simulink model "ADCS_Simulink_FSW"  (R2025b)
settings: Solver=VariableStepAuto  StartTime=8000  StopTime=8700  FixedStep=0.001  RelTol=1e-3
PreLoadFcn:
  | addpath(genpath('../'))
  | adcsModelSetup();
values from neighbouring files (symbols this model uses):
  dT_Control = 1/10    (= 0.1)    [adcsModelSetup.m]
  fNoiseOn = 0    [adcsModelSetup.m]
undefined symbols (not defined in the file or in its folder): DiscIntNeverNeededParam, IAU, juliandate
libraries: vrlib x16, simulink_extras x7, sharedtransform x5, sharedutil x4, aerolibutil x4, sFunctionLibrary x4, simulink x3, matrix_library x2, aerolibtransform2 x2
(part 2 of 2)

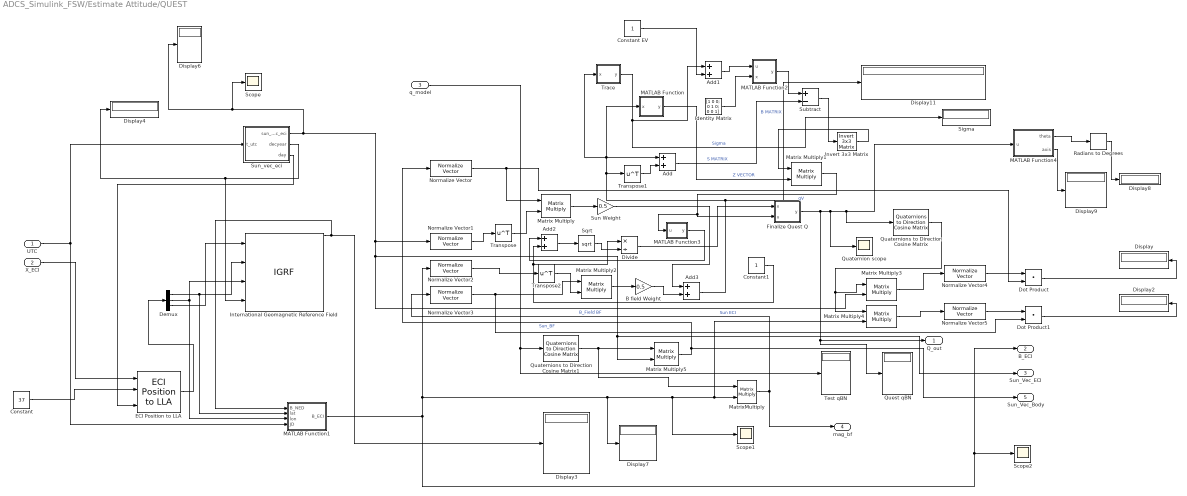
== system ADCS_Simulink_FSW/Estimate Attitude/QUEST ==
  UTC : Inport
  X_ECI : Inport  Port=2
  q_model : Inport  Port=3
  Add{,1..3} (4 alike) : Sum
  B field Weight : Gain  Gain=0.5
  Constant : Constant  Value=37
  Constant EV : Constant
  Constant1 : Constant
  Demux : Demux  Outputs=3
  Display{,2..4,6..9,11} (9 alike) : Display
  Divide : Product  Inputs=*/
  Dot Product : DotProduct  OutDataTypeStr=Inherit: Inherit via internal rule
  Dot Product1 : DotProduct  OutDataTypeStr=Inherit: Inherit via internal rule
  ECI Position to LLA : aerolibtransform2/ECI Position to LLA  red=IAU-2000/2006  year=2013  month=January  day=1  hour=0  min=0  sec=0  deltaT=Day  errorflag=Error  extraparamflag=on  eunits=Metric (MKS)  earthmodel=WGS84  flat=1/298.257223563  eqradius=6378137
      settings: AttributesFormatString=%<red>
  Finalize Quest Q : MATLAB Function  TreatAsAtomicUnit=on
  Identity Matrix : Constant  Value=[1 0 0; 0 1 0; 0 0 1]
  International Geomagnetic Reference Field : IGRF  month=January  day=1  year=2020
      settings: AttributesFormatString=%<generation>
  Invert 3x3 Matrix : aerolibutil/Invert  3x3 Matrix
  MATLAB Function : MATLAB Function  TreatAsAtomicUnit=on
  MATLAB Function1 : MATLAB Function  TreatAsAtomicUnit=on
  MATLAB Function2 : MATLAB Function  TreatAsAtomicUnit=on
  MATLAB Function3 : MATLAB Function  TreatAsAtomicUnit=on
  MATLAB Function4 : MATLAB Function  TreatAsAtomicUnit=on
  Matrix Multiply{,1..5} (6 alike) : Product  Multiplication=Matrix(*)
  MatrixMultiply : Product  Multiplication=Matrix(*)
  Normalize Vector{,1..5} (6 alike) : vrlib/Utilities/Normalize Vector  maxzero=0
  Quaternion scope : Scope
      settings: ActiveDisplayYMinimum=-1.3373181480846994  ActiveDisplayYMaximum=1.336803706475939
  Quaternions to Direction Cosine Matrix : sharedtransform/Quaternions to  Direction Cosine Matrix  aMode=aMode
  Quaternions to Direction Cosine Matrix1 : sharedtransform/Quaternions to  Direction Cosine Matrix  aMode=aMode
  Quest qBN : Display
  Radians to Degrees : simulink_extras/Transformations/Radians to Degrees
  Scope : Scope
      settings: ActiveDisplayYMinimum=-1.0754499109455182  ActiveDisplayYMaximum=0.0072133154143029787
  Scope1 : Scope
      settings: ActiveDisplayYMinimum=-1  ActiveDisplayYMaximum=1  DataLoggingVariableName=ScopeData2
  Scope2 : Scope
      settings: ActiveDisplayYMinimum=-2220.8584339639051  ActiveDisplayYMaximum=7667.7859361134633  DataLoggingVariableName=ScopeData26
  Sigma : Display
  Sqrt : Sqrt
  Subtract : Sum  Inputs=+-
  Sun Weight : Gain  Gain=0.5
  Sun_vec_eci : MATLAB Function  TreatAsAtomicUnit=on
  Test qBN : Display
  Trace : MATLAB Function  TreatAsAtomicUnit=on
  Transpose : Math  Operator=transpose
  Transpose1 : Math  Operator=transpose
  Transpose2 : Math  Operator=transpose
  Q_out : Outport
  B_ECI : Outport  Port=2
  Sun_Vec_ECI : Outport  Port=3
  mag_bf : Outport  Port=4
  Sun_Vec_Body : Outport  Port=5
  wires:
  Sun_vec_eci/3(day) -> ECI Position to LLA/6
  MATLAB Function4/1(theta) -> Radians to Degrees/1
  Finalize Quest Q/1(y) -> Quest qBN/1, Q_out/1, MATLAB Function4/1(u), Quaternions to Direction Cosine Matrix/1, Quaternion scope/1
  Normalize Vector4/1 -> Dot Product/1
  Normalize Vector3/1 -> Matrix Multiply2/1, Dot Product1/2
  Transpose2/1 -> Matrix Multiply2/2
  Normalize Vector1/1 -> Transpose/1
  Normalize Vector5/1 -> Dot Product1/1
  ECI Position to LLA/1 -> Demux/1
  Constant/1 -> ECI Position to LLA/3
  Constant1/1 -> Add2/2, Divide/1
  q_model/1 -> Quaternions to Direction Cosine Matrix1/1, Test qBN/1
  Dot Product/1 -> Display/1
  Sun_vec_eci/1(sun_vec_eci) -> Display6/1, Scope/1, Sun_Vec_ECI/1, Matrix Multiply5/2, Matrix Multiply3/2, Normalize Vector1/1  "Sun ECI"
  Matrix Multiply/1 -> Sun Weight/1
  Demux/1 -> International Geomagnetic Reference Field/2, MATLAB Function1/2(lat)
  Radians to Degrees/1 -> Display8/1
  MatrixMultiply/1 -> Normalize Vector3/1, mag_bf/1  "B_Field BF"
  Quaternions to Direction Cosine Matrix/1 -> Matrix Multiply4/1, Matrix Multiply3/1
  Matrix Multiply5/1 -> Sun_Vec_Body/1, Normalize Vector/1  "Sun_BF"
  Invert 3x3 Matrix/1 -> Matrix Multiply1/1
  Sqrt/1 -> Divide/2
  Demux/3 -> International Geomagnetic Reference Field/1
  Transpose/1 -> Matrix Multiply/2
  Transpose1/1 -> Add/2
  Identity Matrix/1 -> MATLAB Function2/2(x)
  Matrix Multiply3/1 -> Normalize Vector4/1
  Quaternions to Direction Cosine Matrix1/1 -> MatrixMultiply/1, Matrix Multiply5/1
  International Geomagnetic Reference Field/1 -> MATLAB Function1/1(B_NED), Display3/1
  Dot Product1/1 -> Display2/1
  Subtract/1 -> Invert 3x3 Matrix/1
  UTC/1 -> Sun_vec_eci/1(t_utc), MATLAB Function1/4(JD)
  Demux/2 -> MATLAB Function1/3(lon), International Geomagnetic Reference Field/3
  Matrix Multiply2/1 -> B field Weight/1
  Trace/1(y) -> Sigma/1, Add1/1  "Sigma"
  Add/1 -> Subtract/2  "S MATRIX"
  Add2/1 -> Sqrt/1
  MATLAB Function/1(y) -> Matrix Multiply1/2  "Z VECTOR"
  Divide/1 -> Finalize Quest Q/1(x)
  Sun_vec_eci/2(decyear) -> Display4/1, International Geomagnetic Reference Field/4
  Matrix Multiply1/1 -> MATLAB Function3/1(u), Finalize Quest Q/2(u)  "qV"
  X_ECI/1 -> ECI Position to LLA/1
  MATLAB Function2/1(y) -> Subtract/1
  Sun Weight/1 -> Add3/1
  MATLAB Function4/2(axis) -> Display9/1
  Matrix Multiply4/1 -> Normalize Vector5/1
  B field Weight/1 -> Add3/2
  Normalize Vector2/1 -> Transpose2/1
  Add3/1 -> Display11/1, Transpose1/1, MATLAB Function/1(x), Trace/1(x), Add/1  "B MATRIX"
  Add1/1 -> MATLAB Function2/1(u)
  MATLAB Function3/1(y) -> Add2/1
  Normalize Vector/1 -> Matrix Multiply/1, Dot Product/2
  Constant EV/1 -> Add1/2
  MATLAB Function1/1(B_ECI) -> Normalize Vector2/1, MatrixMultiply/2, Matrix Multiply4/2, Scope1/1, Display7/1, Scope2/1, B_ECI/1

== system ADCS_Simulink_FSW/Estimate Attitude/WhiteNoise ==
  Band-Limited White Noise : simulink/Sources/Band-Limited White Noise  Cov=NoisePower  Ts=dT  seed=randi([0 1000],size(NoisePower))
  Data Type Conversion6 : DataTypeConversion  OutDataTypeStr=single  SaturateOnIntegerOverflow=off  RndMeth=Floor
  Out1 : Outport
  wires:
  Band-Limited White Noise/1 -> Data Type Conversion6/1
  Data Type Conversion6/1 -> Out1/1

== system ADCS_Simulink_FSW/NoiseAndDiscretise/GaussianNoise ==
  Data Type Conversion6 : DataTypeConversion  OutDataTypeStr=single  SaturateOnIntegerOverflow=off  RndMeth=Floor
  Random Number : RandomNumber  Mean=Mean  Variance=Variance  Seed=randi([0 1000],size(Variance))  SampleTime=dT  VectorParams1D=off
  Out1 : Outport
  wires:
  Random Number/1 -> Data Type Conversion6/1
  Data Type Conversion6/1 -> Out1/1

== matlab function ADCS_Simulink_FSW/Angle Error ==
  data: u input; y output
function y = fcn(u)
    a = u(1);
    
    y = 2 * acos(a);
end

== matlab function ADCS_Simulink_FSW/Create Desired Quaternion/Calc Angle ==
  data: u input; angle output
function angle = fcn(u)

angle=acos((trace(u)-1)/2);

== matlab function ADCS_Simulink_FSW/Create Desired Quaternion/Calc Axis of rotation ==
  data: a input; y output; b input
function y = fcn(a,b)

y = 1/(2*sin(a))*[b(3,2)-b(2,3); b(1,3)-b(3,1); b(2,1)-b(1,2)];

== matlab function ADCS_Simulink_FSW/Estimate Attitude/QUEST/MATLAB Function ==
  data: x input; y output
function y = fcn(x)
y=ones(3,1);
y(1)=x(2,3)-x(3,2);
y(2)=x(3,1)-x(1,3);
y(3)=x(1,2)-x(2,1);

== matlab function ADCS_Simulink_FSW/Estimate Attitude/QUEST/Finalize Quest Q ==
  data: x input; u input; y output
function y = fcn(x,u)

%x is a scalar, u is the 3x1 vector


q=x*[1;u];
y=q/norm(q);
if y(1)<0
    y = -y;
 end

== matlab function ADCS_Simulink_FSW/Estimate Attitude/QUEST/MATLAB Function2 ==
  data: u input; y output; x input
function y = fcn(u,x)

y=ones(3,3);
y = u*x;

== matlab function ADCS_Simulink_FSW/Estimate Attitude/QUEST/MATLAB Function3 ==
  data: u input; y output
function y = fcn(u)

y = (norm(u))^2;

== matlab function ADCS_Simulink_FSW/Estimate Attitude/Create Quaternion matrix ==
  data: w input; Omega output
function Omega = fcn(w)

wx = w(1); wy = w(2); wz = w(3);

Omega = [ 0   -wx  -wy  -wz;
          wx   0    wz  -wy;
          wy  -wz   0    wx;
          wz   wy  -wx   0  ];

== matlab function ADCS_Simulink_FSW/Estimate Attitude/QUEST/MATLAB Function4 ==
  data: u input; theta output; axis output
function [theta,axis] = fcn(u)
if u(1) < 0
    u = -u; % flip quaternion
end

a = u(1);
theta=2*acos(a);

if abs(sin(theta/2)) < 1e-12
    axis = [0;0;0]; 
else
    axis = u(2:4)/sin(theta/2);
end

== matlab function ADCS_Simulink_FSW/Simulate Omega Rates/Wheel Torque ==
  data: wheel_speeds input; mag_bf input; GsValues input; L_R input; us output; tauMTB output; t_3axis output
function [us, tauMTB,t_3axis]  = f(wheel_speeds, mag_bf, GsValues, L_R)
% MATLAB Function block version of WheelTorque_Command
%
% Inputs:
%   wheel_speeds [4x1]   : Reaction wheel speeds [rad/s]
%   mag_bf       [3x1]   : Magnetic field vector in body frame [T]
%   GsValues     [3x4]   : Wheel geometry / spin axis matrix
%   L_R_input    [3x1]   : Desired control torque from PD controller [Nm]
%
% Output:
%   out_u [7x1] : [us(4x1); tauMTB(3x1)]

    % Constants
    Iws = 0.000029382450521;   % Wheel spin axis inertia [kg·m^2]
    c   = 0.025;                % Reaction wheel torque to magtorquer scaler
    OmegaD = rpm_to_rads(250) * ones(4,1);  % Desired wheel bias [rad/s]

    % Wheel speed vector
    Omega = wheel_speeds(:);

    % L_R from PD controller
    L_R = L_R(:);

    % Torque rod transformation (identity)
    Gt = eye(3);

    % Compute pseudo-inverse of Gs
    Gs = GsValues;
    Gs_pinv = pinv(Gs);

    % RW torque required to track commanded torque
    usReq = Gs_pinv * (-L_R);  %usReq is a 4 by 1 quantity

    % Despin torque
    usStar = -c * Iws * (Omega - OmegaD);

    % Skew-symmetric matrix of magnetic field
    B_tilde = [   0      -mag_bf(3)  mag_bf(2);
               mag_bf(3)     0      -mag_bf(1);
              -mag_bf(2)  mag_bf(1)     0     ];

     
    Btilde_Gt = B_tilde * Gt;
    muStar = -pinv(Btilde_Gt) * Gs * usStar;
    for i = 1:3
        if(muStar(i)>.1)
            muStar(i) = .1;
        end
        if(muStar(i)<-.1)
            muStar(i) = -.1;
        end
    end

    % Magnetic torque
    tauMTB = -(Btilde_Gt) * muStar;

    % deltaU = pinv(Gs) * (tauMTB - Gs*usStar)
    deltaU = Gs_pinv * (tauMTB - Gs * usStar);

    % Actual applied RW torque
    us = usReq + usStar + deltaU;

    for i = 1:4
        if(us(i)>.0032)
        us(i) = .0032;
        end
        if(us(i)<-.0032)
        us(i)=-.0032;
        end
    end

    t_3axis = -Gs*us;

end

% Helper: RPM to rad/s
function rad_s = rpm_to_rads(rpm)
    rad_s = rpm * (2*pi/60);
end

== matlab function ADCS_Simulink_FSW/Single Axis Error/Compute single axis rotation ==
  data: a input; y output; b input
function y = fcn(a, b)

axis = cross(a, b);
axis_norm = norm(axis);

if axis_norm < 1e-8
    if dot(a,b) > 0   %Vectors is parallel
        y = [1; 0; 0; 0];

    else              %Vectors are antiparallel
        axis = null(a(:).');
        axis = axis(:,1)/norm(axis(:,1));
        y = [0; axis];
    end
    return
end

axis = cross(a, b);
axis_norm = norm(axis);
axis = axis / axis_norm;
angle = acos(dot(a, b) / (norm(a)*norm(b)));

y = zeros(4,1);
y(1) = cos(angle / 2);
y(2:4) = axis * sin(angle / 2);

% if(y(1)<0)
%     y=-y;
% end

== matlab function ADCS_Simulink_FSW/Estimate Attitude/QUEST/MATLAB Function1 ==
  data: B_NED input; B_ECI output; lat input; lon input; JD input
function B_ECI = ned2eci(B_NED, lat, lon, JD)
% Converts magnetic field vector from NED to ECI
% Inputs:
%   B_NED = [Bn; Be; Bd] magnetic field vector in NED [any units]
%   lat, lon = geodetic latitude, longitude [deg]
%   JD = Julian Date
% Output:
%   B_ECI = [Bx; By; Bz] in ECI coordinates [same units]

lon = deg2rad(lon);
lat = deg2rad(lat);
% ----- 1. Compute GMST -----
JD0 = floor(JD + 0.5) - 0.5;
H = (JD - JD0) * 24;             % hours since 0h UT
D = JD - 2451545.0;
D0 = JD0 - 2451545.0;
T = D / 36525;

GMST_hours = 6.697374558 + 0.06570982441908 * D0 + 1.00273790935 * H + 0.000026 * T^2;
GMST_hours = mod(GMST_hours, 24);         % wrap 0-24h
theta_g = deg2rad(15 * GMST_hours);       % convert to radians

% ----- 2. Rotation from NED -> ECEF -----
R_ECEF_NED = [ -sin(lat)*cos(lon), -sin(lat)*sin(lon),  cos(lat);
               -sin(lon),            cos(lon),           0;
               -cos(lat)*cos(lon),  -cos(lat)*sin(lon), -sin(lat) ];

% ----- 3. Rotation from ECEF -> ECI -----
R_ECI_ECEF = [ cos(theta_g), -sin(theta_g), 0;
               sin(theta_g),  cos(theta_g), 0;
               0,              0,           1 ];

% ----- 4. Combine rotations -----
B_ECI = R_ECI_ECEF * R_ECEF_NED * B_NED;
end

== matlab function ADCS_Simulink_FSW/Simulate Omega Rates/Clamp WS ==
  data: u input; y output
function y = fcn(u)

max_threshold=6500*((2*pi)/60);
min_threshold=120*((2*pi)/60);

for i=1:4
if(u(i)>max_threshold)
    u(i)=max_threshold;
elseif(u(i)<-min_threshold)
    u(i)=-min_threshold;
end

end
y=u;

== matlab function ADCS_Simulink_FSW/Create Desired Quaternion/DCOMM & CSAC/MATLAB Function ==
  data: JD_now input; day output
function day = fcn(JD_now)

baseJD_start =  2.460950250000000e+06;
day = JD_now - baseJD_start;

== matlab function ADCS_Simulink_FSW/Angle Error1 ==
  data: u input; y output
function y = fcn(u)
    a = u(1);
    
    y = 2 * acos(a);
end

== matlab function ADCS_Simulink_FSW/Estimate Attitude/QUEST/Sun_vec_eci ==
  data: sun_vec_eci output; decyear output; day output; t_utc input
function [sun_vec_eci, decyear, day] = SunVecECI_codegen(t_utc)
% Codegen-safe function for Simulink
% Input: t_utc (Julian Date)
% Outputs:
%   sun_vec_eci - 3x1 Sun unit vector in ECI
%   decyear     - decimal year (for IGRF)
%   day         - day of month (for IGRF)

% --- Constants ---
JD_J2000 = 2451545.0; % reference JD for 2000-01-01 12:00 UTC

% --- Compute approximate year ---
days_since_2000 = t_utc - JD_J2000;
year = 2000 + floor(days_since_2000 / 365.25);

% --- Compute day-of-year fraction ---
JD_start_of_year = JD_J2000 + (year-2000)*365.25; % approximate start of year
frac_day_of_year = t_utc - JD_start_of_year;

% --- Compute day of month (simplified for IGRF) ---
% approximate: 12 months = 365.25/12 ~ 30.4375 days per month
day = floor(mod(frac_day_of_year, 30.4375)) + 1;

% --- Decimal year ---
decyear = year + frac_day_of_year / 365.25;

% --- Clamp for IGRF ---
if decyear > 2025
    decyear = 2025;
elseif decyear < 1900
    decyear = 1900;
end

% --- Sun vector in ECI ---
D_days = t_utc - JD_J2000; % days since J2000
g = 357.529 + 0.98560028 * D_days;           
q = 280.459 + 0.98564736 * D_days;          
L = q + 1.914666471*sind(g) + 0.018994643*sind(2*g);
e = 23.439291 - 0.0130042*(D_days/36525); 

x = cosd(L);
y = cosd(e)*sind(L);
z = sind(e)*sind(L);
 sun_vec_eci = [x; y; z];
% sun_vec_eci= [-0.9672; 4; -0.10];

end

== matlab function ADCS_Simulink_FSW/Create Desired Quaternion/Check Flippage ==
  data: u input; y output
function y = fcn(u)

y = u;
if(u(1)<0)
y=-u;
end

== matlab function ADCS_Simulink_FSW/Estimate Attitude/QUEST/Trace ==
  data: x input; y output
function y = fcn(x)

y=x(1,1)+x(2,2)+x(3,3);

== matlab function ADCS_Simulink_FSW/Angle Error2 ==
  data: u input; y output
function y = fcn(u)
    a = u(1);
    
    y = 2 * acos(a);
end

== matlab function ADCS_Simulink_FSW/Estimate Attitude/buildBk ==
  data: magVec input single; y output single size=[3 2]; sunVec input single
function y = combineMagSunMeas(magVec,sunVec)
    
    y = single(zeros(3,2));
    y(:,1) = magVec;
    y(:,2) = sunVec;
end

== matlab function ADCS_Simulink_FSW/Estimate Attitude/buildEci_k ==
  data: magVec input single; y output single size=[3 2]; sunVec input single
function y = combineMagSunMeas(magVec,sunVec)
    
    y = single(zeros(3,2));
    y(:,1) = magVec;
    y(:,2) = sunVec;
end

== matlab function ADCS_Simulink_FSW/Estimate Attitude/Angle Error2 ==
  data: u input; y output
function y = fcn(u)
    a = u(1);
    
    y = 2 * acos(a);
end

== matlab function ADCS_Simulink_FSW/Create Desired Quaternion/Singularity Fix(Sheppards Method) ==
  data: q input; y output
function y = fcn(q)

% y=q;
% if(q(1)<1e-2)
C = quat2dcm_passive(q);
t = trace(C);

p0 = 0.25*(1+t);
p1 = 0.25*(1 + (2*C(1,1)) - t);
p2 = 0.25*(1 + (2*C(2,2)) - t);
p3 = 0.25*(1 + (2*C(3,3)) - t);

[maxv,idx] = max([p0, p1, p2, p3]);
if(idx==1)
b0=sqrt(maxv);
b1 = (C(2,3) - C(3,2))/(4*b0);
b2 = (C(3,1) - C(1,3))/(4*b0);
b3 = (C(1,2) - C(2,1))/(4*b0);

elseif(idx==2)
b1 = sqrt(maxv);
b0 = (C(2,3) - C(3,2))/(4*b1);
b2 = (C(1,2) + C(2,1))/(4*b1);
b3 = (C(3,1) + C(1,3))/(4*b1);

elseif(idx == 3)
b2 = sqrt(maxv);
b0 = (C(3,1) - C(1,3))/(4*b2);
b1 = (C(1,2) + C(2,1))/(4*b2);
b3 = (C(2,3) + C(3,2))/(4*b2);

else
 b3 = sqrt(maxv);
 b0 = (C(1,2) - C(2,1))/(4*b3);
 b1 = (C(3,1) + C(1,3))/(4*b3);
 b2 = (C(2,3) + C(3,2))/(4*b3);
end

y = [b0;b1;b2;b3];

% end

 if(y(1)<0)
        y=-y;
 end

end
function C = quat2dcm_passive(q)
% q = [q0 q1 q2 q3]'  (scalar-first, Hamilton)
% Passive quaternion -> DCM (coordinate transformation)

q = q(:);
q = q / norm(q);   % ensure unit quaternion

q0 = q(1); q1 = q(2); q2 = q(3); q3 = q(4);

C = [ ...
    q0^2+q1^2-q2^2-q3^2,   2*(q1*q2+q0*q3),       2*(q1*q3-q0*q2);
    2*(q1*q2-q0*q3),       q0^2-q1^2+q2^2-q3^2,   2*(q2*q3+q0*q1);
    2*(q1*q3+q0*q2),       2*(q2*q3-q0*q1),       q0^2-q1^2-q2^2+q3^2 ...
    ];
end

== matlab function ADCS_Simulink_FSW/Estimate Attitude/Check Flippage ==
  data: u input; y output
function y = fcn(u)

if u(1)<0
     y = -u;
else 
    y=u;
end

== matlab function ADCS_Simulink_FSW/Create Desired Quaternion/create DCM ==
  data: y output; dv input; v1 output; v2 output; doter output; unitx input
function [y,v1,v2,doter]  = fcn(dv,unitx)
% unitx=[1; 0; 0];
unity=[0; 1; 0];


doter=abs(dot(dv,unitx));

if(doter<0.99)
v1=cross(dv,unitx);

else %if parallel
v1=cross(dv,unity);
end

v1=v1/norm(v1);
v2=cross(dv,v1);
v2=v2/norm(v2);

y=[dv,v1,v2];
determinant = det(y);


end

== matlab function ADCS_Simulink_FSW/Create Desired Quaternion/DCOMM & CSAC/Determine best GS ==
  data: y output; pos_ecef input; bdangle output; best output
function [y, bdangle,best]= fcn(pos_ecef)

gnd_stat = [  -1286433.52, -4720122.48, 4079330.11;   % Ground Station 1 - Denver, USA
               3875201.89,   87312.44, 5025191.62;    % Ground Station 2 - London, UK
              -2476842.13,  4678921.75, -3556211.38;  % Ground Station 3 - Perth, Australia
               1112103.57, -6123457.23, 1210234.99 ]; % Ground Station 4 - Santiago, Chile

smallest = inf;
best=0;
bdangle=50;  %just a filler
for i=1:4
        gnd=gnd_stat(i,:);
  
        gs2sc=pos_ecef-gnd';
        distance=norm(gs2sc);
        zenrad=acos(dot(gs2sc,gnd)/(norm(gs2sc)*norm(gnd)));
        zenangle=rad2deg(zenrad);
       if zenangle<90
            if distance<smallest
                smallest=distance;
                best=i;
                bdangle=zenangle;
            end
       end
end
if best == 0
y=zeros(3,1);
% disp("Yo we got zeroes");
else
y=gnd_stat(best,:)';
end

== matlab function ADCS_Simulink_FSW/PD Controller/Calculate Error ==
  data: q1 input; q output; q2 input
function q = fcn(q1, q2)
% MATLAB IMPLEMENTATION

    w1 = q1(1); x1 = q1(2); y1 = q1(3); z1 = q1(4);
    w2 = q2(1); x2 = q2(2); y2 = q2(3); z2 = q2(4);

    w = w1*w2 - x1*x2 - y1*y2 - z1*z2;
    x = w1*x2 + x1*w2 + y1*z2 - z1*y2;
    y = w1*y2 - x1*z2 + y1*w2 + z1*x2;
    z = w1*z2 + x1*y2 - y1*x2 + z1*w2;

    q = [w; x; y; z];
    q=q/norm(q);

    % if(q(1)<0)
    %  q=-q;
    % end

% COPYING FLIGHT CODE

end

== matlab function ADCS_Simulink_FSW/Create Desired Quaternion/Mode Switch ==
  data: c input; y output; sv input; sc2gs input; phicone input; t input; dc input
function y = fcn(c,sv,sc2gs,phicone,t,dc)

% if(t>=200)
% c=3
% end
% if (t>400)
% c=2
% end

if c==1
y=sv;
elseif c==2
    if norm(dc)==0 
    y=sv;
    else
    y=sc2gs;
    end
elseif c==3
y=phicone;
else
y=sv;
end

== matlab function ADCS_Simulink_FSW/Calculate Desired Rates/Angle betwen 2 vec ==
  data: a input; y output; b input
function y = fcn(a,b)

val = dot(a,b)/(norm(a)*norm(b));
val = max(-1, min(1, val));
y = acos(val);

== matlab function ADCS_Simulink_FSW/Create Desired Quaternion/DCOMM & CSAC/final phicone vec ==
  data: svec input; y output; zenith input
function y = fcn(svec,zenith)

y = cosd(45)*zenith + sind(45)*svec;
y=y/norm(y);

== matlab function ADCS_Simulink_FSW/Simulate Omega Rates/Gravity Gradient Torque ==
  data: J input; Tgg output; pos_bf input
function Tgg = fcn(J, pos_bf)

mag=norm(pos_bf);
u_const=3.986004418e14;
u_bf=pos_bf/mag;


coef=3*u_const/(mag^3);
t1=J*u_bf;
init=cross(u_bf,t1);
Tgg=coef*init;
